simulink model "ADRCliju"  (R2024b)
settings: Solver=FixedStepAuto  StartTime=0.0  StopTime=20  RelTol=1e-3
undefined symbols (not defined in the file or in its folder): sigbuilder_block
libraries: spsPermanentMagnetSynchronousMachineLib x2, slpidlib x2, simulink x2, powerlib_extras x2, Solver_SF x1, spsDCVoltageSourceLib x1, spsUniversalBridgeLib x1, spspowerguiLib x1
settings Model: Creator=Dell  LastModifiedBy=L大锤
settings SolverCC: AlgebraicLoopSolver=TrustRegion
settings DataIOCC: ReturnWorkspaceOutputs=off
settings DebuggingCC: UnconnectedInputMsg=warning  UnconnectedOutputMsg=warning  UnconnectedLineMsg=warning  ArithmeticOperatorsInVariantConditions=warning
settings ModelReferenceCC: EnableRefExpFcnMdlSchedulingChecks=on
settings SFSimCC: CustomCodeUndefinedFunction=UseInterfaceOnly
settings RTWCC: GPUComputeCapability=3.5

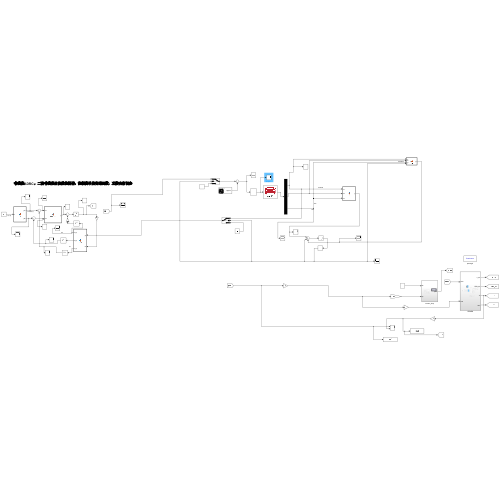
[thumbnail: Simulink's stored preview of the top-level diagram]
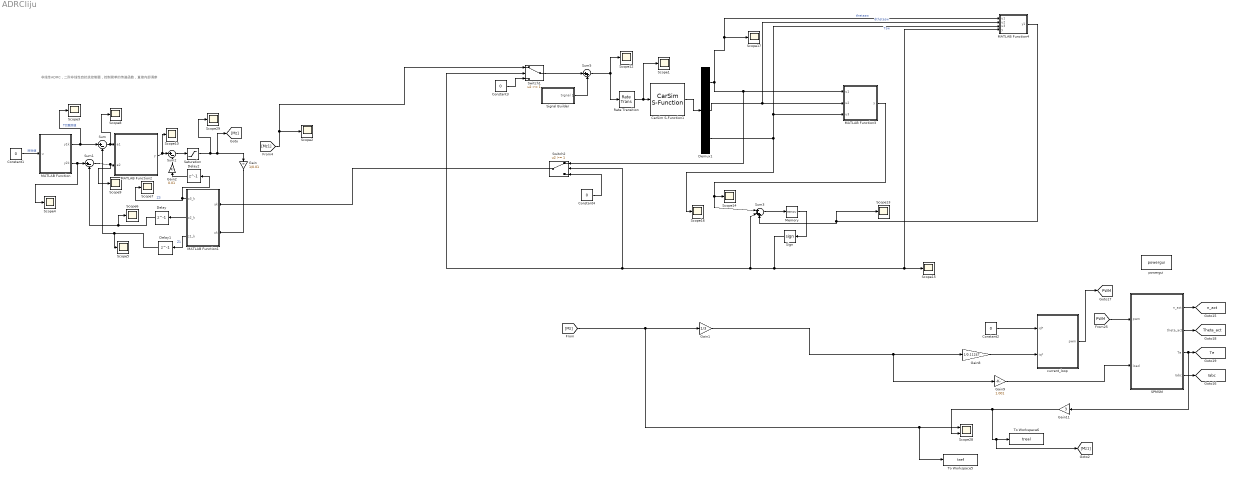
== system ADRCliju ==
  note: 非线性ADRC，二阶非线性自抗扰控制器，控制简单的传递函数，直接内部调参
  CarSim S-Function1 : Solver_SF/CarSim S-Function  Priority=1  SIMFILE=simfile.sim  Run_RTs=off  vs_state_ind=Run  StopMode_ind=Vehicle Model
  Constant{1..4} (4 alike) : Constant  Value=0
  Delay : Delay  DelayLength=1
  Delay1 : Delay  DelayLength=1
  Delay2 : Delay  DelayLength=1
  Demux1 : Demux  Outputs=3
  Gain : Gain  Gain=1/0.01
  Gain1 : Gain  Gain=1/3
  Gain11 : Gain  Gain=3
  Gain2 : Gain  Gain=0.01
  Gain8 : Gain  Gain=1/0.11247
  Gain9 : Gain  Gain=1.001
  MATLAB Function : MATLAB Function  TreatAsAtomicUnit=on
  MATLAB Function1 : MATLAB Function  TreatAsAtomicUnit=on
  MATLAB Function2 : MATLAB Function  TreatAsAtomicUnit=on
  MATLAB Function3 : MATLAB Function  TreatAsAtomicUnit=on
  MATLAB Function4 : MATLAB Function  TreatAsAtomicUnit=on
  Memory : Memory
  Rate Transition : RateTransition  OutPortSampleTime=1e-5
  SPMSM : Subsystem
  Saturation : Saturate  UpperLimit=2.99  LowerLimit=-2.99
  Scope{1..10,12..17,29} (17 alike) : Scope
  Scope28 : Scope  NumInputPorts=2
  Sign : Signum
  Signal Builder : Subsystem  Tag=STV Subsys  LoadFcn=sigbuilder_block('load');  StartFcn=sigbuilder_block('start');  StopFcn=sigbuilder_block('stop');  ClipboardFcn=sigbuilder_block('clipboard');  mask(Sigbuilder block){tuvar=[0:10]}
      mask help: Simulink:masks:SigbuilderBlock_MD
      mask init:
      | if ~strcmp(get_param(bdroot(gcbh),'SimulationStatus'),'stopped') tuvar = sigbuilder_block('maskInit'); end
      settings: CopyFcn=sigbuilder_block('copy');  DeleteFcn=sigbuilder_block('delete');  ModelCloseFcn=sigbuilder_block('modelClose');  PreSaveFcn=sigbuilder_block('preSave');  PauseFcn=sigbuilder_block('pause');  ContinueFcn=sigbuilder_block('continue');  NameChangeFcn=sigbuilder_block('namechange');  OpenFcn=sigbuilder_block('open',[437.6 186.6 550.4 400.2 ]);  CloseFcn=sigbuilder_block('close');
      mask Display: plot(0, 0, 100, 100,[2, 2, 32, 32, 2], [68, 8, 8, 68, 68],[32, 2], [38, 38], [32, 19, 2],[53, 60, 44], [32, 17, 17, 2],[16, 16, 31, 31]);txt = getActiveGroup(gcbh);text(2, 100, txt,'verticalAlignment', 'top');
  Sum : Sum  Inputs=|+-
  Sum1 : Sum  Inputs=|+-
  Sum2 : Sum  Inputs=|+-
  Sum3 : Sum  Inputs=|+++
  Sum5 : Sum  Inputs=|++
  Switch1 : Switch  Threshold=1  SaturateOnIntegerOverflow=off  InputSameDT=off
  Switch2 : Switch  Threshold=1  SaturateOnIntegerOverflow=off  InputSameDT=off
  To Workspace5 : ToWorkspace  VariableName=tref  SampleTime=-1
  To Workspace6 : ToWorkspace  VariableName=treal  SampleTime=-1
  current_loop : Subsystem
  powergui : spspowerguiLib/powergui  Priority=1  SimulationMode=Continuous  SampleTime=1/2000/500  frequency=60  Iterations=50  frequencyindice=0  Pbase=100e6  ErrMax=1e-4  UnitsV=kV  UnitsW=MW  buscounter=0  FunctionMessages=off  echomessages=off  EnableUseOfTLC=off  CurrentSourceSwitches=off  DisableSnubberDevices=off  DisableRonSwitches=off  DisableVfSwitches=off  DisplayEquations=off  AutomaticDiscreteSolvers=off  SolverType=Tustin/Backward Euler (TBE)  Interpol=off  ExternalGateDelay=off  methode=off  Ts=100  x0status=blocks  SPID=on  SwTol=0  HookPort=off  NonlinearTolerance=1e-4  nMaxIteration=100  ContinueOnMaxIteration=off  RestoreLinks=warning  ResistiveCurrentMeasurement=off  Frange=[0:2:500]  Ylog=off  Xlog=on  ShowGrid=off  save=off  variable=ZData  structure=ia  ZoomFFT=off  StartTime=.775  cycles=1  DisplayStyle=1  fundamental=400  FreqAxis=off  MaxFrequency=40000  frequencyindicesteady=1  RmsSteady=1  display=off
  tag scope: Iabc=global, PWM=global, Te=global, Theta_act=global, n_act=global
  wires:
  Constant1/1 -> MATLAB Function/1(u)  "目标值"
  Sum/1 -> Scope8/1, MATLAB Function2/1(e1)
  MATLAB Function/2(y2k) -> Scope4/1, Sum1/1
  Sum1/1 -> Scope9/1, MATLAB Function2/2(e2)
  MATLAB Function/1(y1k) -> Scope3/1, Sum/1  "TD跟踪值"
  Gain2/1 -> Sum2/2
  MATLAB Function1/1(z3_k) -> Scope7/1, Delay2/1  "Z3"
  MATLAB Function2/1(y) -> Scope10/1, Sum2/1
  Gain/1 -> MATLAB Function1/2(uk)
  MATLAB Function1/2(z2_k) -> Delay/1
  Delay/1 -> Scope6/1, Sum1/2
  Delay2/1 -> Gain2/1
  MATLAB Function1/3(z1_k) -> Delay1/1  "Z1"
  Delay1/1 -> Scope5/1, Sum/2
  Sum2/1 -> Saturation/1
  Saturation/1 -> Scope29/1, Gain/1, [Mz]
  [Mz] -> To Workspace5/1, Scope28/1, Gain1/1
  SPMSM/3(Te) -> Gain11/1, [Te]
  SPMSM/1(n_act) -> [n_act]
  [PWM] -> SPMSM/1(pwm)
  Constant2/1 -> current_loop/1(id*)
  Gain9/1 -> SPMSM/2(load)
  Gain8/1 -> current_loop/2(iq*)
  Gain11/1 -> [Mz1], To Workspace6/1, Scope28/2
  current_loop/1(pwm) -> [PWM]
  SPMSM/2(theta_act) -> [Theta_act]
  SPMSM/4(Iabc) -> [Iabc]
  Gain1/1 -> Gain9/1, Gain8/1
  Signal Builder/1(Signal 1) -> Sum5/2
  Switch2/1 -> MATLAB Function1/1(yk)
  CarSim S-Function1/1 -> Demux1/1
  Constant4/1 -> Switch2/3
  Sum5/1 -> Rate Transition/1, Scope12/1
  MATLAB Function3/1(y) -> Sum3/1, Scope14/1
  Demux1/1 -> Scope17/1, MATLAB Function4/1(u1), Switch2/1, MATLAB Function3/1(u1)  "thetasw"
  [Mz1] -> Switch1/1, Scope2/1
  Sign/1 -> Switch1/2, Switch2/2, Sum3/2, MATLAB Function4/4(y), Scope15/1
  Sum3/1 -> Memory/1
  MATLAB Function4/1(y1) -> Scope13/1, Sum3/3
  Demux1/2 -> MATLAB Function4/2(u2), MATLAB Function3/2(u2)  "dthstasw"
  Constant3/1 -> Switch1/3
  Memory/1 -> Sign/1
  Switch1/1 -> Sum5/1
  Demux1/3 -> MATLAB Function3/3(u3), MATLAB Function4/3(u3), Scope16/1  "Tsw"
  Rate Transition/1 -> CarSim S-Function1/1, Scope1/1

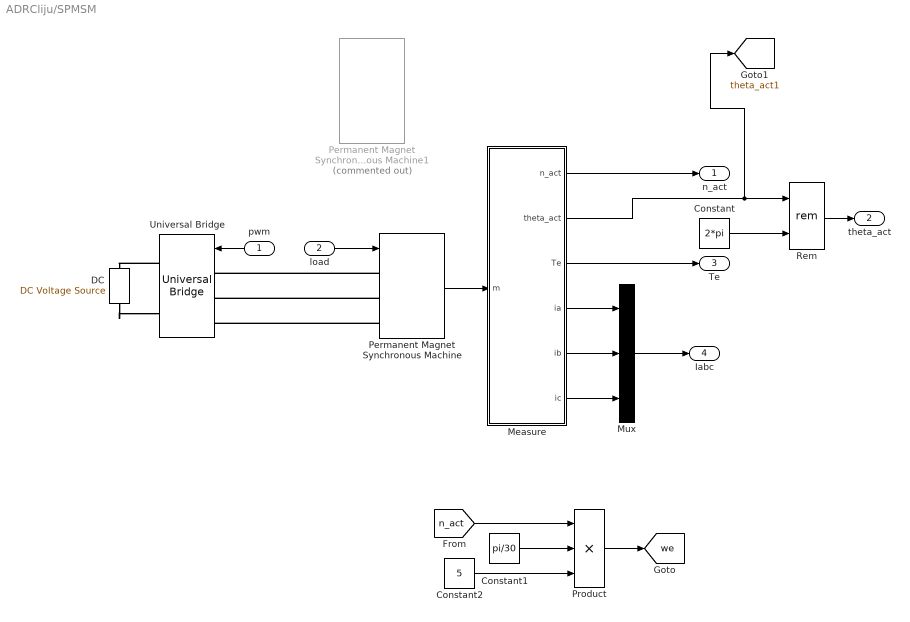
== system ADRCliju/SPMSM ==
  pwm : Inport
  load : Inport  Port=2
  Constant : Constant  Value=2*pi
  Constant1 : Constant  Value=pi/30
  Constant2 : Constant  Value=5
  "DC " : spsDCVoltageSourceLib/DC Voltage Source  Amplitude=200  Measurements=None
  Measure : Subsystem
  Mux : Mux  Inputs=3
  Permanent Magnet Synchronous Machine : spsPermanentMagnetSynchronousMachineLib/Permanent Magnet Synchronous Machine  NbPhases=3  FluxDistribution=Sinusoidal  RotorType=Round  MechanicalLoad=Torque Tm  PresetModel=No  ShowDetailedParameters=on  MeasurementBus=off  Resistance=0.12  Inductance=8.5e-3  dqInductances=[4e-3, 4e-3]  La=0.97e-3  MachineConstant=Voltage Constant (V_peak L-L / krpm)  Flux=0.014996  VoltageCst=13.6  TorqueCst=0.11247  Flat=120  Mechanical=[0.00107 0 5 0]  PolePairs=4  InitialConditions=[0,0, 0,0]  InitialConditions5ph=[0 0 0 0 0 0]  RefAngle=Aligned with phase A axis (original Park)  IterativeDiscreteModel=Trapezoidal non iterative  TsBlock=-1  TsPowergui=0
  Permanent Magnet Synchronous Machine1 : spsPermanentMagnetSynchronousMachineLib/Permanent Magnet Synchronous Machine  Commented=on  NbPhases=3  FluxDistribution=Sinusoidal  RotorType=Salient-pole  MechanicalLoad=Torque Tm  PresetModel=No  ShowDetailedParameters=on  MeasurementBus=off  Resistance=2.875  Inductance=8.5e-3  dqInductances=[4e-3, 4e-3]  La=0.000835  MachineConstant=Flux linkage established by magnets (V.s)  Flux=0.175  VoltageCst=126.966  TorqueCst=1.05  Flat=120  Mechanical=[0.003 0 4 0]  PolePairs=4  InitialConditions=[0,0, 0,0]  InitialConditions5ph=[0 0 0 0 0 0]  RefAngle=Aligned with phase A axis (original Park)  IterativeDiscreteModel=Trapezoidal non iterative  TsBlock=-1  TsPowergui=0
  Product : Product  Inputs=3
  Rem : Math  Operator=rem
  Universal Bridge : spsUniversalBridgeLib/Universal Bridge  Arms=3  SnubberResistance=1e5  SnubberCapacitance=inf  Device=IGBT / Diodes  Ron=1e-3  Lon=0  ForwardVoltages="[  0  0  ]"  ForwardVoltage=0  GTOparameters=[ 10e-6 , 20e-6 ]  IGBTparameters=[ 1e-6 , 2e-6 ]  Measurements=None  Measurements_2=None  converterType=Rectifier
  n_act : Outport
  theta_act : Outport  Port=2
  Te : Outport  Port=3
  Iabc : Outport  Port=4
  tag scope: theta_act1=global, we=global
  wires:
  pwm/1 -> Universal Bridge/1
  load/1 -> Permanent Magnet Synchronous Machine/1
  Permanent Magnet Synchronous Machine/1 -> Measure/1(m)
  Measure/1(n_act) -> n_act/1
  Measure/3(Te) -> Te/1
  Measure/4(ia) -> Mux/1
  Measure/5(ib) -> Mux/2
  Measure/6(ic) -> Mux/3
  Mux/1 -> Iabc/1
  Rem/1 -> theta_act/1
  Constant/1 -> Rem/2
  Measure/2(theta_act) -> [theta_act1], Rem/1
  [n_act] -> Product/1
  Constant1/1 -> Product/2
  Constant2/1 -> Product/3
  Product/1 -> [we]
  connections:
  "DC "/LConn1 -- Universal Bridge/RConn2
  Universal Bridge/RConn1 -- "DC "/RConn1
  Permanent Magnet Synchronous Machine/LConn3 -- Universal Bridge/LConn3
  Permanent Magnet Synchronous Machine/LConn1 -- Universal Bridge/LConn1
  Permanent Magnet Synchronous Machine/LConn2 -- Universal Bridge/LConn2

== system ADRCliju/Signal Builder ==
  Demux : Demux  Tag=STV Demux  Outputs=1
      settings: DisplayOption=none
  FromWs : FromWorkspace  Tag=STV FromWs  VariableName=tuvar
      SigBuilderData=|
      | common.afterFinalStr = 'Extrapolate'
      | common.sampleTime = 0
      | dataSet.timeRange = [0 10]
      | dataSet.name = 'Group 1'
      | sbobj.Groups.Name = 'Group 1'
      | sbobj.Groups.Signals.Name = 'Signal 1'
      | sbobj.Groups.Signals.XData = [0 1 1 5 5 10]
      | sbobj.Groups.Signals.YData = [0 0 4 4 0 0]
  Signal 1 : Outport  Tag=STV Outport
  wires:
  Demux/1 -> Signal 1/1
  FromWs/1 -> Demux/1

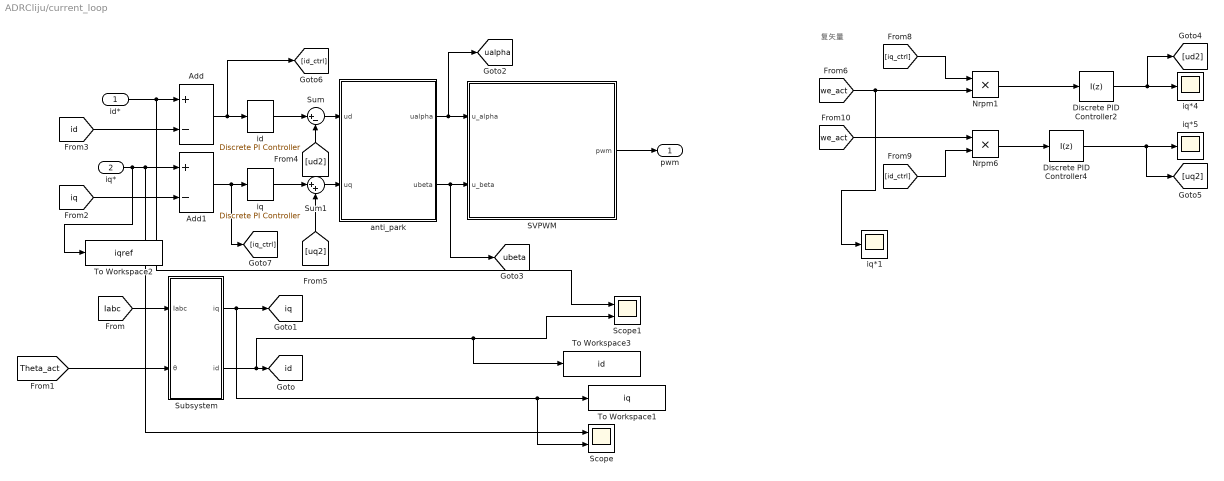
== system ADRCliju/current_loop ==
  note: 复矢量
  id* : Inport
  iq* : Inport  Port=2
  Add : Sum  Inputs=+-
  Add1 : Sum  Inputs=+-
  Discrete PID Controller2 : slpidlib/PID Controller  Controller=I  Form=Parallel  TimeDomain=Discrete-time  UseExternalTs=off  SampleTime=1e-4  IntegratorMethod=Forward Euler  FilterMethod=Forward Euler  ControllerParametersSource=internal  P=0  I=0.32/10000  UseKiTs=off  D=0  UseExternalDerivativeSource=off  N=100  UseFilter=on  TunerSelectOption=Transfer Function Based (PID Tuner App)  InitialConditionSource=internal  InitialConditionForIntegrator=0  InitialConditionForFilter=0  DifferentiatorICPrevScaledInput=0  ExternalReset=none  TrackingMode=off  Kt=1  LimitOutput=on  SatLimitsSource=internal  UpperSaturationLimit=600  LowerSaturationLimit=-600  LinearizeAsGain=off  AntiWindupMode=none  Kb=1  LimitIntegrator=off  UpperIntegratorSaturationLimit=inf  LowerIntegratorSaturationLimit=-inf  POutMin=[]  POutMax=[]  IOutMin=[]  IOutMax=[]  DOutMin=[]  DOutMax=[]  NOutMin=[]  NOutMax=[]  SumOutMin=[]  SumOutMax=[]  SaturationOutMin=[]  SaturationOutMax=[]  PParamMin=[]  PParamMax=[]  IParamMin=[]  IParamMax=[]  DParamMin=[]  DParamMax=[]  NParamMin=[]  NParamMax=[]  KbParamMin=[]  KbParamMax=[]  KtParamMin=[]  KtParamMax=[]  KbOutMin=[]  KbOutMax=[]  KtOutMin=[]  KtOutMax=[]  IntegratorOutMin=[]  IntegratorOutMax=[]  FilterOutMin=[]  FilterOutMax=[]  SumI1OutMin=[]  SumI1OutMax=[]  SumI2OutMin=[]  SumI2OutMax=[]  SumI3OutMin=[]  SumI3OutMax=[]  SumI4OutMin=[]  SumI4OutMax=[]  SumDOutMin=[]  SumDOutMax=[]  DifferentiatorOutMin=[]  DifferentiatorOutMax=[]  FilterDiffOutCoefMin=[]  FilterDiffOutCoefMax=[]  ReciprocalOutMin=[]  ReciprocalOutMax=[]  SumDenOutMin=[]  SumDenOutMax=[]  SumNumOutMin=[]  SumNumOutMax=[]  DivideOutMin=[]  DivideOutMax=[]  UdiffTsProdOutMin=[]  UdiffTsProdOutMax=[]  NTsProdOutMin=[]  NTsProdOutMax=[]  UintegralTsProdOutMin=[]  UintegralTsProdOutMax=[]  UngainTsProdOutMin=[]  UngainTsProdOutMax=[]  ClampingZeroOutDataTypeStr=Inherit: Inherit via back propagation  ClampingZeroOutMin=[]  ClampingZeroOutMax=[]  FilterDenConstantOutDataTypeStr=Inherit: Inherit via back propagation  FilterDenConstantOutMin=[]  FilterDenConstantOutMax=[]  PCopyOutDataTypeStr=Inherit: Inherit via back propagation  PCopyOutMin=[]  PCopyOutMax=[]  NCopyOutDataTypeStr=Inherit: Inherit via back propagation  NCopyOutMin=[]  NCopyOutMax=[]  IntegratorContinuousStateAttributes=''  IntegratorStateMustResolveToSignalObject=off  IntegratorRTWStateStorageClass=Auto  FilterContinuousStateAttributes=''  FilterStateMustResolveToSignalObject=off  FilterRTWStateStorageClass=Auto  ParallelPVariant=Disabled  IdealPVariant=Disabled  IVariant=InternalParameters  DVariant=Disabled  IntegratorVariant=Discrete  SatVariant=Enabled  AWVariant=Passthrough  PCopyVariant=Disabled  TRVariant=Disabled  FdbkBlocksVariant=Forward  IdealPFdbkVariant=Disabled  SatFdbkVariant=Disabled  DerivativeFilterVariant=Disabled  NVariant=Disabled  NCopyVariant=Disabled_SignalSpec  FilterICVariant=Disabled  IntegratorICVariant=InternalICs  ExternalResetVariant=Disabled  TRSumVariant=Passthrough  SumFdbkVariant=Disabled  SumVariant=Passthrough_I  TsampFilterVariant=InternalTs  TsampNgainVariant=Passthrough  TsampIntegralVariant=Disabled_SignalSpec  ExternalSaturationOutDataTypeStr=Inherit: Same as second input  DerivativeSourceVariant=Disabled  PreIntVariant=InternalPreInt
  Discrete PID Controller4 : slpidlib/PID Controller  Controller=I  Form=Parallel  TimeDomain=Discrete-time  UseExternalTs=off  SampleTime=1e-4  IntegratorMethod=Forward Euler  FilterMethod=Forward Euler  ControllerParametersSource=internal  P=0  I=0.32/10000  UseKiTs=off  D=0  UseExternalDerivativeSource=off  N=100  UseFilter=on  TunerSelectOption=Transfer Function Based (PID Tuner App)  InitialConditionSource=internal  InitialConditionForIntegrator=0  InitialConditionForFilter=0  DifferentiatorICPrevScaledInput=0  ExternalReset=none  TrackingMode=off  Kt=1  LimitOutput=on  SatLimitsSource=internal  UpperSaturationLimit=600  LowerSaturationLimit=-600  LinearizeAsGain=off  AntiWindupMode=none  Kb=1  LimitIntegrator=off  UpperIntegratorSaturationLimit=inf  LowerIntegratorSaturationLimit=-inf  POutMin=[]  POutMax=[]  IOutMin=[]  IOutMax=[]  DOutMin=[]  DOutMax=[]  NOutMin=[]  NOutMax=[]  SumOutMin=[]  SumOutMax=[]  SaturationOutMin=[]  SaturationOutMax=[]  PParamMin=[]  PParamMax=[]  IParamMin=[]  IParamMax=[]  DParamMin=[]  DParamMax=[]  NParamMin=[]  NParamMax=[]  KbParamMin=[]  KbParamMax=[]  KtParamMin=[]  KtParamMax=[]  KbOutMin=[]  KbOutMax=[]  KtOutMin=[]  KtOutMax=[]  IntegratorOutMin=[]  IntegratorOutMax=[]  FilterOutMin=[]  FilterOutMax=[]  SumI1OutMin=[]  SumI1OutMax=[]  SumI2OutMin=[]  SumI2OutMax=[]  SumI3OutMin=[]  SumI3OutMax=[]  SumI4OutMin=[]  SumI4OutMax=[]  SumDOutMin=[]  SumDOutMax=[]  DifferentiatorOutMin=[]  DifferentiatorOutMax=[]  FilterDiffOutCoefMin=[]  FilterDiffOutCoefMax=[]  ReciprocalOutMin=[]  ReciprocalOutMax=[]  SumDenOutMin=[]  SumDenOutMax=[]  SumNumOutMin=[]  SumNumOutMax=[]  DivideOutMin=[]  DivideOutMax=[]  UdiffTsProdOutMin=[]  UdiffTsProdOutMax=[]  NTsProdOutMin=[]  NTsProdOutMax=[]  UintegralTsProdOutMin=[]  UintegralTsProdOutMax=[]  UngainTsProdOutMin=[]  UngainTsProdOutMax=[]  ClampingZeroOutDataTypeStr=Inherit: Inherit via back propagation  ClampingZeroOutMin=[]  ClampingZeroOutMax=[]  FilterDenConstantOutDataTypeStr=Inherit: Inherit via back propagation  FilterDenConstantOutMin=[]  FilterDenConstantOutMax=[]  PCopyOutDataTypeStr=Inherit: Inherit via back propagation  PCopyOutMin=[]  PCopyOutMax=[]  NCopyOutDataTypeStr=Inherit: Inherit via back propagation  NCopyOutMin=[]  NCopyOutMax=[]  IntegratorContinuousStateAttributes=''  IntegratorStateMustResolveToSignalObject=off  IntegratorRTWStateStorageClass=Auto  FilterContinuousStateAttributes=''  FilterStateMustResolveToSignalObject=off  FilterRTWStateStorageClass=Auto  ParallelPVariant=Disabled  IdealPVariant=Disabled  IVariant=InternalParameters  DVariant=Disabled  IntegratorVariant=Discrete  SatVariant=Enabled  AWVariant=Passthrough  PCopyVariant=Disabled  TRVariant=Disabled  FdbkBlocksVariant=Forward  IdealPFdbkVariant=Disabled  SatFdbkVariant=Disabled  DerivativeFilterVariant=Disabled  NVariant=Disabled  NCopyVariant=Disabled_SignalSpec  FilterICVariant=Disabled  IntegratorICVariant=InternalICs  ExternalResetVariant=Disabled  TRSumVariant=Passthrough  SumFdbkVariant=Disabled  SumVariant=Passthrough_I  TsampFilterVariant=InternalTs  TsampNgainVariant=Passthrough  TsampIntegralVariant=Disabled_SignalSpec  ExternalSaturationOutDataTypeStr=Inherit: Same as second input  DerivativeSourceVariant=Disabled  PreIntVariant=InternalPreInt
  Nrpm1 : Product
  Nrpm6 : Product
  SVPWM : Subsystem
  Scope : Scope  NumInputPorts=2
  Scope1 : Scope  NumInputPorts=2
  Subsystem : Subsystem
  Sum : Sum  Inputs=|+-
  Sum1 : Sum  Inputs=|++
  To Workspace1 : ToWorkspace  VariableName=iq  SampleTime=-1
  To Workspace2 : ToWorkspace  VariableName=iqref  SampleTime=-1
  To Workspace3 : ToWorkspace  VariableName=id  SampleTime=-1
  anti_park : Subsystem
  id : powerlib_extras/Discrete  Control Blocks/Discrete PI Controller  Kp=0.32*2  Ki=0.004*2  Par_Limits=[200/1.732 -200/1.732]  Init=0  Ts=1e-4
  iq : powerlib_extras/Discrete  Control Blocks/Discrete PI Controller  Kp=0.32*2  Ki=0.004*2  Par_Limits=[200/1.732 -200/1.732]  Init=0  Ts=1e-4
  iq*1 : Scope
  iq*4 : Scope
  iq*5 : Scope
  pwm : Outport
  tag scope: id=global, iq=global, ualpha=global, ubeta=global
  wires:
  id*/1 -> Scope1/1, Add/1
  Add/1 -> [id_ctrl], id/1
  iq*/1 -> To Workspace2/1, Scope/1, Add1/1
  Add1/1 -> [iq_ctrl], iq/1
  anti_park/1(ualpha) -> [ualpha], SVPWM/1(u_alpha)
  anti_park/2(ubeta) -> [ubeta], SVPWM/2(u_beta)
  SVPWM/1(pwm) -> pwm/1
  [Iabc] -> Subsystem/1(Iabc)
  [iq] -> Add1/2
  [id] -> Add/2
  [Theta_act] -> Subsystem/2(θ)
  [ud2] -> Sum/2
  [uq2] -> Sum1/2
  id/1 -> Sum/1
  Sum/1 -> anti_park/1(ud)
  iq/1 -> Sum1/1
  Sum1/1 -> anti_park/2(uq)
  [id_ctrl] -> Nrpm6/2
  Nrpm1/1 -> Discrete PID Controller2/1
  Nrpm6/1 -> Discrete PID Controller4/1
  Discrete PID Controller2/1 -> [ud2], iq*4/1
  [we_act] -> iq*1/1, Nrpm1/2
  [we_act] -> Nrpm6/1
  Discrete PID Controller4/1 -> iq*5/1, [uq2]
  [iq_ctrl] -> Nrpm1/1
  Subsystem/2(id) -> To Workspace3/1, Scope1/2, [id]
  Subsystem/1(iq) -> To Workspace1/1, Scope/2, [iq]

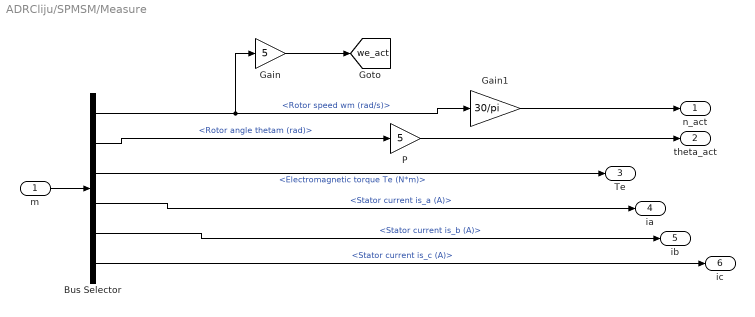
== system ADRCliju/SPMSM/Measure ==
  m : Inport
  Bus Selector : BusSelector  OutputSignals=Rotor speed wm (rad/s),Rotor angle thetam (rad),Electromagnetic torque Te (N*m),Stator current is_a (A),Stator current is_b (A),Stator current is_c (A)
  Gain : Gain  Gain=5
  Gain1 : Gain  Gain=30/pi
  P : Gain  Gain=5
  n_act : Outport  VectorParamsAs1DForOutWhenUnconnected=off
  theta_act : Outport  Port=2  VectorParamsAs1DForOutWhenUnconnected=off
  Te : Outport  Port=3  VectorParamsAs1DForOutWhenUnconnected=off
  ia : Outport  Port=4  VectorParamsAs1DForOutWhenUnconnected=off
  ib : Outport  Port=5  VectorParamsAs1DForOutWhenUnconnected=off
  ic : Outport  Port=6  VectorParamsAs1DForOutWhenUnconnected=off
  tag scope: we_act=global
  wires:
  m/1 -> Bus Selector/1
  Bus Selector/3 -> Te/1  "<Electromagnetic torque Te (N*m)>"
  Bus Selector/1 -> Gain/1, Gain1/1  "<Rotor speed wm (rad/s)>"
  Bus Selector/2 -> P/1  "<Rotor angle thetam (rad)>"
  Bus Selector/5 -> ib/1  "<Stator current is_b (A)>"
  Bus Selector/6 -> ic/1  "<Stator current is_c (A)>"
  P/1 -> theta_act/1
  Gain1/1 -> n_act/1
  Bus Selector/4 -> ia/1  "<Stator current is_a (A)>"
  Gain/1 -> [we_act]

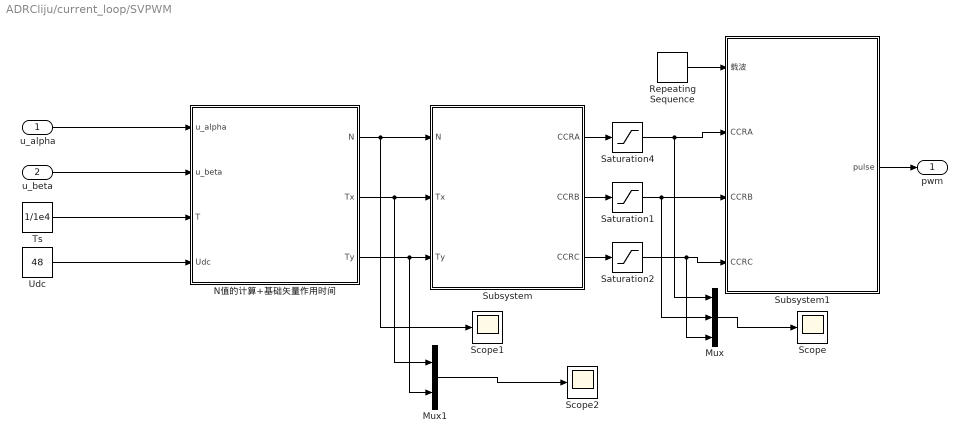
== system ADRCliju/current_loop/SVPWM ==
  u_alpha : Inport
  u_beta : Inport  Port=2
  Mux : Mux  Inputs=3
  Mux1 : Mux  Inputs=2
  N值的计算+基础矢量作用时间 : Subsystem
  Repeating Sequence : simulink/Sources/Repeating Sequence  rep_seq_t=[0 1/1e4/2 1/1e4]  rep_seq_y=[0 1/1e4/2 0]
  Saturation1 : Saturate  UpperLimit=1/1e4/2  LowerLimit=0
  Saturation2 : Saturate  UpperLimit=1/1e4/2  LowerLimit=0
  Saturation4 : Saturate  UpperLimit=1/1e4/2  LowerLimit=0
  Scope : Scope
  Scope1 : Scope
  Scope2 : Scope
  Subsystem : Subsystem
  Subsystem1 : Subsystem
  Ts : Constant  Value=1/1e4
  Udc : Constant  Value=48
  pwm : Outport
  wires:
  Repeating Sequence/1 -> Subsystem1/1(载波)
  Subsystem1/1(pulse) -> pwm/1
  N值的计算+基础矢量作用时间/3(Ty) -> Mux1/2, Subsystem/3(Ty)
  N值的计算+基础矢量作用时间/2(Tx) -> Mux1/1, Subsystem/2(Tx)
  N值的计算+基础矢量作用时间/1(N) -> Scope1/1, Subsystem/1(N)
  Udc/1 -> N值的计算+基础矢量作用时间/4(Udc)
  Ts/1 -> N值的计算+基础矢量作用时间/3(T)
  u_beta/1 -> N值的计算+基础矢量作用时间/2(u_beta)
  u_alpha/1 -> N值的计算+基础矢量作用时间/1(u_alpha)
  Subsystem/2(CCRB) -> Saturation1/1
  Subsystem/3(CCRC) -> Saturation2/1
  Subsystem/1(CCRA) -> Saturation4/1
  Mux/1 -> Scope/1
  Saturation4/1 -> Mux/1, Subsystem1/2(CCRA)
  Saturation1/1 -> Mux/2, Subsystem1/3(CCRB)
  Saturation2/1 -> Mux/3, Subsystem1/4(CCRC)
  Mux1/1 -> Scope2/1

== system ADRCliju/current_loop/Subsystem ==
  Iabc : Inport
  θ : Inport  Port=2
  Clark : Subsystem
  Demux : Demux  Outputs=3
  "Park " : Subsystem
  iq : Outport  VectorParamsAs1DForOutWhenUnconnected=off
  id : Outport  Port=2  VectorParamsAs1DForOutWhenUnconnected=off
  tag scope: ialpha=global, ibeta=global
  wires:
  Demux/1 -> Clark/1(ia)
  Demux/3 -> Clark/3(ic)
  Demux/2 -> Clark/2(ib)
  Iabc/1 -> Demux/1
  θ/1 -> "Park "/3(Theta)
  Clark/2(ibeta) -> [ibeta], "Park "/2(ibeta)
  Clark/1(ialfa) -> [ialpha], "Park "/1(ialfa)
  "Park "/1(iq) -> iq/1
  "Park "/2(id) -> id/1

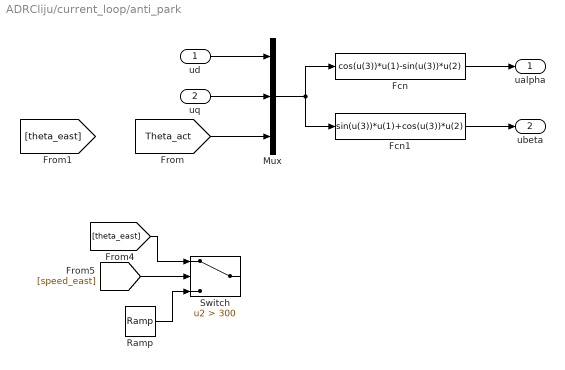
== system ADRCliju/current_loop/anti_park ==
  ud : Inport
  uq : Inport  Port=2
  Fcn : Fcn  Expr=cos(u(3))*u(1)-sin(u(3))*u(2)
  Fcn1 : Fcn  Expr=sin(u(3))*u(1)+cos(u(3))*u(2)
  Mux : Mux  Inputs=3
  Ramp : simulink/Sources/Ramp  slope=50  start=0  InitialOutput=0
  Switch : Switch  Criteria=u2 > Threshold  Threshold=300  SaturateOnIntegerOverflow=off  InputSameDT=off
  ualpha : Outport
  ubeta : Outport  Port=2
  wires:
  Fcn/1 -> ualpha/1
  ud/1 -> Mux/1
  uq/1 -> Mux/2
  Fcn1/1 -> ubeta/1
  Mux/1 -> Fcn/1, Fcn1/1
  [theta_east] -> Switch/1
  Ramp/1 -> Switch/3
  [speed_east] -> Switch/2
  [Theta_act] -> Mux/3

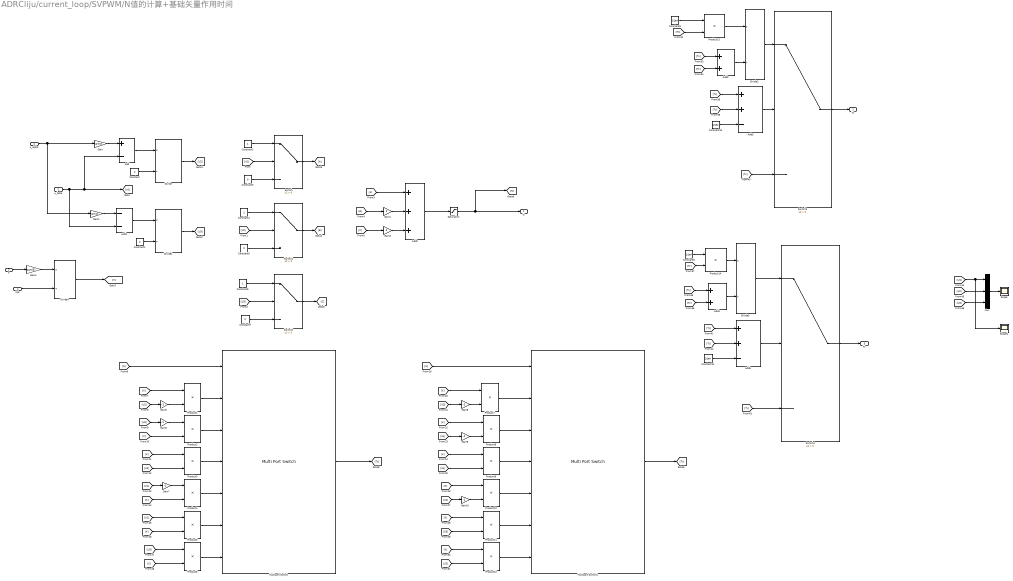
== system ADRCliju/current_loop/SVPWM/N值的计算+基础矢量作用时间 ==
  u_alpha : Inport
  u_beta : Inport  Port=2
  T : Inport  Port=3
  Udc : Inport  Port=4
  Add : Sum  Inputs=+-
  Add1 : Sum  Inputs=--
  Add2 : Sum  Inputs=+++
  Add3 : Sum
  Add4 : Sum
  Add5 : Sum  Inputs=++-
  Add6 : Sum  Inputs=++-
  Constant : Constant  Value=2
  Constant1 : Constant  Value=2
  Constant{8..11} (4 alike) : Constant  Value=1/1e4
  Constant2 : Constant
  Constant3 : Constant  Value=0
  Constant4 : Constant
  Constant5 : Constant  Value=0
  Constant6 : Constant
  Constant7 : Constant  Value=0
  Divide{,1..4} (5 alike) : Product  Inputs=*/
  From3 : From
  Gain : Gain  Gain=sqrt(3)
  Gain1 : Gain  Gain=2
  Gain{5..10} (6 alike) : Gain  Gain=-1
  Gain2 : Gain  Gain=sqrt(3)
  Gain3 : Gain  Gain=4
  Gain4 : Gain  Gain=sqrt(3)
  Goto3 : Goto
  Multiport Switch : MultiPortSwitch  Inputs=6  SaturateOnIntegerOverflow=off  InputSameDT=off
  Multiport Switch1 : MultiPortSwitch  Inputs=6  SaturateOnIntegerOverflow=off  InputSameDT=off
  Mux : Mux  Inputs=3
  Product{1..14} (14 alike) : Product
  Saturation : Saturate  UpperLimit=6  LowerLimit=1
  Scope : Scope
  Scope1 : Scope
  Switch{,1..4} (5 alike) : Switch  Criteria=u2 > Threshold  SaturateOnIntegerOverflow=off  InputSameDT=off
  N : Outport
  Tx : Outport  Port=2
  Ty : Outport  Port=3
  wires:
  Switch4/1 -> Ty/1
  [Ty] -> Switch4/3
  Constant11/1 -> Add6/3
  [Ty] -> Add6/2
  [Tx] -> Add6/1
  Add6/1 -> Switch4/2
  Divide3/1 -> Switch4/1
  Switch3/1 -> Tx/1
  [Tx] -> Switch3/3
  Constant10/1 -> Add5/3
  [Ty] -> Add5/2
  [Tx] -> Add5/1
  Add5/1 -> Switch3/2
  Divide2/1 -> Switch3/1
  [Ty] -> Product14/2
  Constant9/1 -> Product14/1
  Product14/1 -> Divide3/1
  [Tx] -> Add4/1
  [Ty] -> Add4/2
  Add4/1 -> Divide3/2
  [Ty] -> Add3/2
  [Tx] -> Add3/1
  Add3/1 -> Divide2/2
  [Tx] -> Product13/2
  Constant8/1 -> Product13/1
  Product13/1 -> Divide2/1
  [U2] -> Product12/2
  [K] -> Product12/1
  Product12/1 -> Multiport Switch1/7
  [U3] -> Product11/2
  [K] -> Product11/1
  Product11/1 -> Multiport Switch1/6
  Gain10/1 -> Product10/2
  [U2] -> Gain10/1
  [K] -> Product10/1
  Product10/1 -> Multiport Switch1/5
  [U1] -> Product9/2
  [K] -> Product9/1
  Product9/1 -> Multiport Switch1/4
  Gain9/1 -> Product8/2
  [U1] -> Gain9/1
  [K] -> Product8/1
  Product8/1 -> Multiport Switch1/3
  Multiport Switch1/1 -> [Ty]
  Gain8/1 -> Product7/2
  [U3] -> Gain8/1
  [K] -> Product7/1
  Product7/1 -> Multiport Switch1/2
  [N] -> Multiport Switch1/1
  [K] -> Product6/2
  [U3] -> Product6/1
  Product6/1 -> Multiport Switch/7
  [K] -> Product5/2
  [U1] -> Product5/1
  Product5/1 -> Multiport Switch/6
  [K] -> Product4/2
  [U1] -> Gain7/1
  Gain7/1 -> Product4/1
  Product4/1 -> Multiport Switch/5
  [U2] -> Product3/2
  [K] -> Product3/1
  Product3/1 -> Multiport Switch/4
  [K] -> Product2/2
  Gain6/1 -> Product2/1
  [U3] -> Gain6/1
  Gain5/1 -> Product1/2
  Product2/1 -> Multiport Switch/3
  Multiport Switch/1 -> [Tx]
  [U2] -> Gain5/1
  [K] -> Product1/1
  Product1/1 -> Multiport Switch/2
  Udc/1 -> Divide4/2
  T/1 -> Gain4/1
  Gain4/1 -> Divide4/1
  Divide4/1 -> [K]
  [N] -> Multiport Switch/1
  Saturation/1 -> N/1, [N]
  Add2/1 -> Saturation/1
  [C] -> Gain3/1
  Gain3/1 -> Add2/3
  [B] -> Gain1/1
  Gain1/1 -> Add2/2
  From3/1 -> Add2/1
  Switch2/1 -> [C]
  Constant7/1 -> Switch2/3
  Constant6/1 -> Switch2/1
  [U3] -> Switch2/2
  Switch1/1 -> [B]
  Constant5/1 -> Switch1/3
  Constant4/1 -> Switch1/1
  [U2] -> Switch1/2
  Constant3/1 -> Switch/3
  Constant2/1 -> Switch/1
  Switch/1 -> Goto3/1
  [U1] -> Switch/2
  u_beta/1 -> [U1], Add/2, Add1/2
  Gain2/1 -> Add1/1
  Divide1/1 -> [U3]
  Constant1/1 -> Divide1/2
  Add1/1 -> Divide1/1
  Divide/1 -> [U2]
  Constant/1 -> Divide/2
  Add/1 -> Divide/1
  u_alpha/1 -> Gain/1, Gain2/1
  Gain/1 -> Add/1
  [U1] -> Scope1/1, Mux/1
  [U2] -> Mux/2
  [U3] -> Mux/3
  Mux/1 -> Scope/1

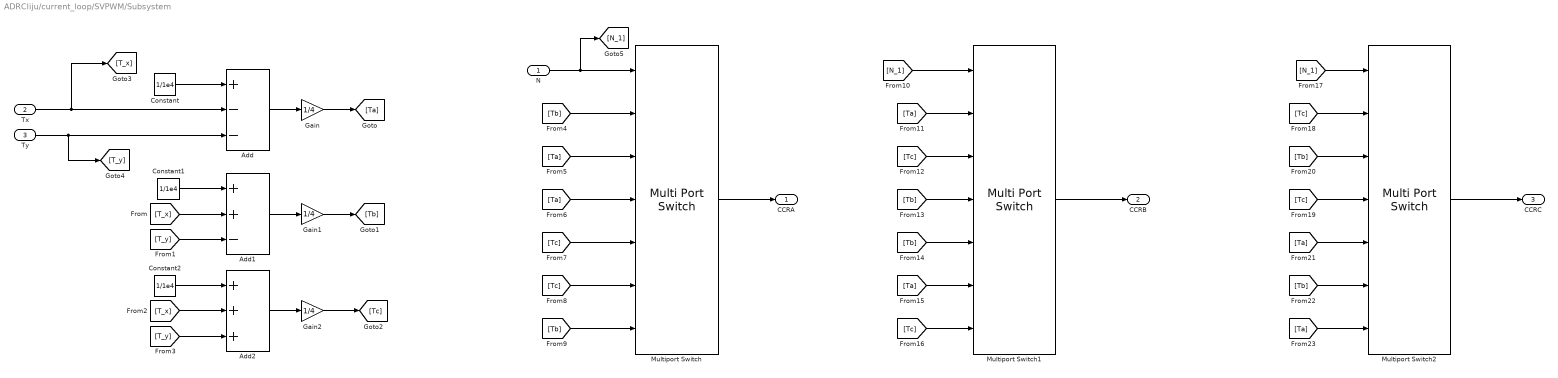
== system ADRCliju/current_loop/SVPWM/Subsystem ==
  N : Inport
  Tx : Inport  Port=2
  Ty : Inport  Port=3
  Add : Sum  Inputs=+--
  Add1 : Sum  Inputs=++-
  Add2 : Sum  Inputs=+++
  Constant : Constant  Value=1/1e4
  Constant1 : Constant  Value=1/1e4
  Constant2 : Constant  Value=1/1e4
  Gain : Gain  Gain=1/4
  Gain1 : Gain  Gain=1/4
  Gain2 : Gain  Gain=1/4
  Multiport Switch : MultiPortSwitch  Inputs=6  SaturateOnIntegerOverflow=off  InputSameDT=off
  Multiport Switch1 : MultiPortSwitch  Inputs=6  SaturateOnIntegerOverflow=off  InputSameDT=off
  Multiport Switch2 : MultiPortSwitch  Inputs=6  SaturateOnIntegerOverflow=off  InputSameDT=off
  CCRA : Outport
  CCRB : Outport  Port=2
  CCRC : Outport  Port=3
  wires:
  [Ta] -> Multiport Switch2/7
  [Tb] -> Multiport Switch2/6
  [Ta] -> Multiport Switch2/5
  [Tc] -> Multiport Switch2/4
  [Tb] -> Multiport Switch2/3
  [Tc] -> Multiport Switch2/2
  Multiport Switch2/1 -> CCRC/1
  [N_1] -> Multiport Switch2/1
  [Tc] -> Multiport Switch1/7
  [Ta] -> Multiport Switch1/6
  [Tb] -> Multiport Switch1/5
  [Tb] -> Multiport Switch1/4
  [Tc] -> Multiport Switch1/3
  [Ta] -> Multiport Switch1/2
  Multiport Switch1/1 -> CCRB/1
  [N_1] -> Multiport Switch1/1
  [Tb] -> Multiport Switch/7
  [Tc] -> Multiport Switch/6
  [Tc] -> Multiport Switch/5
  [Ta] -> Multiport Switch/4
  [Ta] -> Multiport Switch/3
  [Tb] -> Multiport Switch/2
  Multiport Switch/1 -> CCRA/1
  N/1 -> Multiport Switch/1, [N_1]
  [T_y] -> Add2/3
  [T_x] -> Add2/2
  Constant2/1 -> Add2/1
  Gain2/1 -> [Tc]
  Add2/1 -> Gain2/1
  Gain1/1 -> [Tb]
  Add1/1 -> Gain1/1
  [T_y] -> Add1/3
  [T_x] -> Add1/2
  Constant1/1 -> Add1/1
  Gain/1 -> [Ta]
  Add/1 -> Gain/1
  Ty/1 -> Add/3, [T_y]
  Tx/1 -> Add/2, [T_x]
  Constant/1 -> Add/1

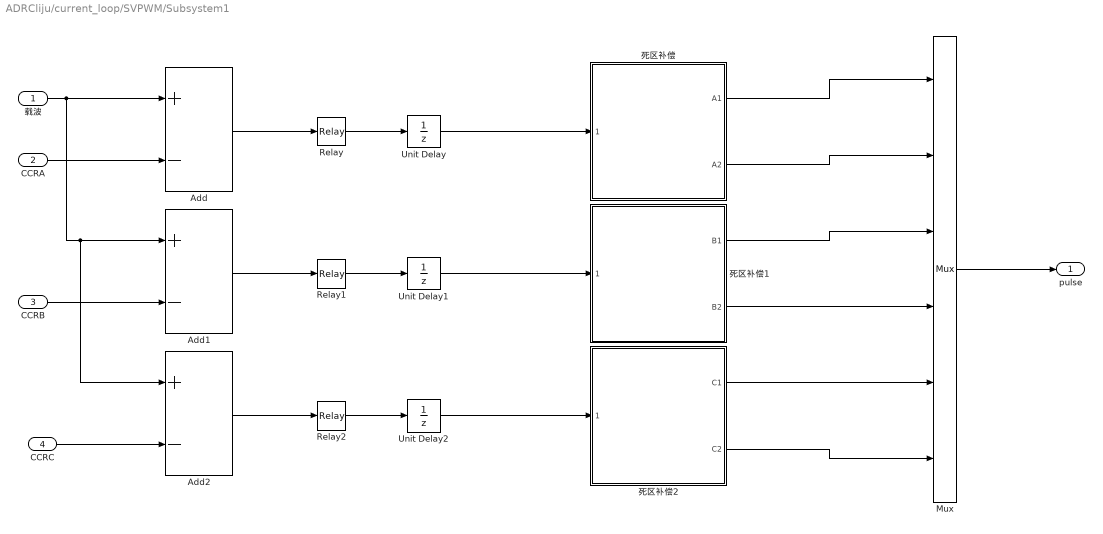
== system ADRCliju/current_loop/SVPWM/Subsystem1 ==
  载波 : Inport
  CCRA : Inport  Port=2
  CCRB : Inport  Port=3
  CCRC : Inport  Port=4
  Add : Sum  Inputs=+-
  Add1 : Sum  Inputs=+-
  Add2 : Sum  Inputs=+-
  Mux : Mux  Inputs=6
  Relay : Relay
  Relay1 : Relay
  Relay2 : Relay
  Unit Delay : UnitDelay  SampleTime=-1  HasFrameUpgradeWarning=on
  Unit Delay1 : UnitDelay  SampleTime=-1  HasFrameUpgradeWarning=on
  Unit Delay2 : UnitDelay  SampleTime=-1  HasFrameUpgradeWarning=on
  死区补偿 : Subsystem
  死区补偿1 : Subsystem
  死区补偿2 : Subsystem
  pulse : Outport
  wires:
  Mux/1 -> pulse/1
  死区补偿2/2(C2) -> Mux/6
  死区补偿2/1(C1) -> Mux/5
  死区补偿1/2(B2) -> Mux/4
  死区补偿1/1(B1) -> Mux/3
  死区补偿/2(A2) -> Mux/2
  死区补偿/1(A1) -> Mux/1
  Unit Delay2/1 -> 死区补偿2/1(1)
  Unit Delay1/1 -> 死区补偿1/1(1)
  Unit Delay/1 -> 死区补偿/1(1)
  Relay2/1 -> Unit Delay2/1
  Relay1/1 -> Unit Delay1/1
  Relay/1 -> Unit Delay/1
  Add2/1 -> Relay2/1
  Add1/1 -> Relay1/1
  Add/1 -> Relay/1
  CCRC/1 -> Add2/2
  CCRB/1 -> Add1/2
  CCRA/1 -> Add/2
  载波/1 -> Add/1, Add1/1, Add2/1

== system ADRCliju/current_loop/Subsystem/Clark ==
  ia : Inport
  ib : Inport  Port=2
  ic : Inport  Port=3
  Fcn : Fcn  Expr=2/3*(u[1]-0.5*u[2]-0.5*u[3])
  Fcn1 : Fcn  Expr=2/3*(sqrt(3/4)*u(2)-sqrt(3/4)*u(3))
  Mux : Mux  Inputs=3
  ialfa : Outport  VectorParamsAs1DForOutWhenUnconnected=off
  ibeta : Outport  Port=2  VectorParamsAs1DForOutWhenUnconnected=off
  wires:
  ic/1 -> Mux/3
  Fcn1/1 -> ibeta/1
  Fcn/1 -> ialfa/1
  Mux/1 -> Fcn1/1, Fcn/1
  ib/1 -> Mux/2
  ia/1 -> Mux/1

== system ADRCliju/current_loop/Subsystem/Park  ==
  ialfa : Inport
  ibeta : Inport  Port=2
  Theta : Inport  Port=3
  Fcn : Fcn  Expr=u(2)*cos(u(3))-u(1)*sin(u(3))
  Fcn1 : Fcn  Expr=u(2)*sin(u(3))+u(1)*cos(u(3))
  Mux : Mux  Inputs=3
  iq : Outport  VectorParamsAs1DForOutWhenUnconnected=off
  id : Outport  Port=2  VectorParamsAs1DForOutWhenUnconnected=off
  wires:
  Theta/1 -> Mux/3
  Fcn1/1 -> id/1
  Fcn/1 -> iq/1
  Mux/1 -> Fcn/1, Fcn1/1
  ibeta/1 -> Mux/2
  ialfa/1 -> Mux/1

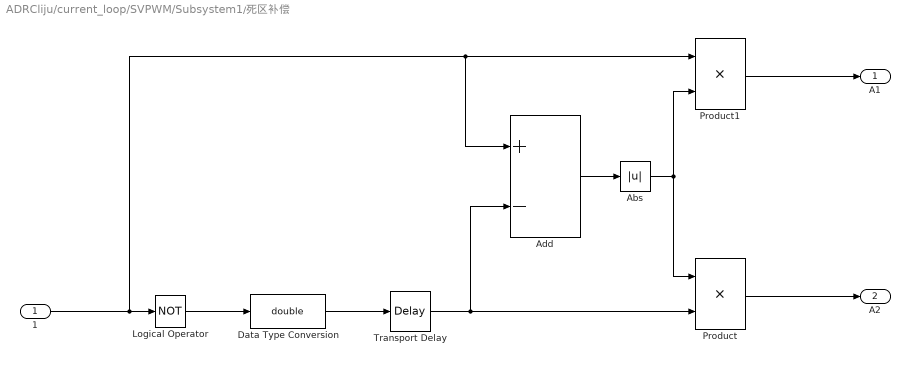
== system ADRCliju/current_loop/SVPWM/Subsystem1/死区补偿 ==
  1 : Inport
  Abs : Abs  SaturateOnIntegerOverflow=off
  Add : Sum  Inputs=+-
  Data Type Conversion : DataTypeConversion  OutDataTypeStr=double  SaturateOnIntegerOverflow=off  RndMeth=Floor
  Logical Operator : Logic  Operator=NOT  AllPortsSameDT=off  OutDataTypeStr=boolean
  Product : Product
  Product1 : Product
  Transport Delay : TransportDelay  DelayTime=0
  A1 : Outport
  A2 : Outport  Port=2
  wires:
  Abs/1 -> Product1/2, Product/1
  Product1/1 -> A1/1
  Add/1 -> Abs/1
  Product/1 -> A2/1
  Transport Delay/1 -> Product/2, Add/2
  Data Type Conversion/1 -> Transport Delay/1
  Logical Operator/1 -> Data Type Conversion/1
  1/1 -> Logical Operator/1, Add/1, Product1/1

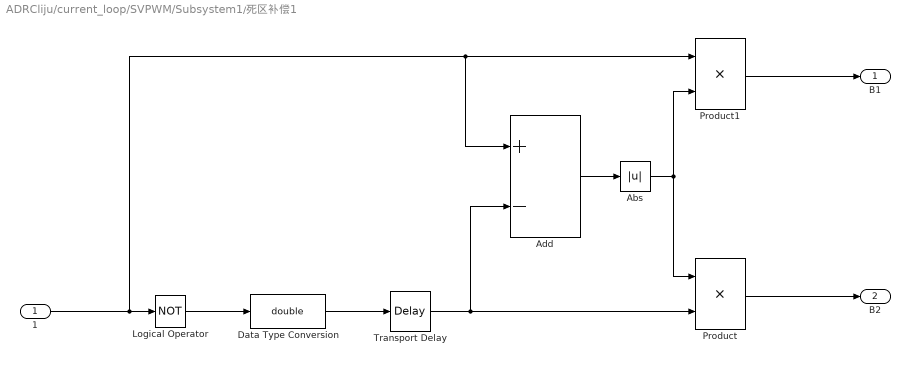
== system ADRCliju/current_loop/SVPWM/Subsystem1/死区补偿1 ==
  1 : Inport
  Abs : Abs  SaturateOnIntegerOverflow=off
  Add : Sum  Inputs=+-
  Data Type Conversion : DataTypeConversion  OutDataTypeStr=double  SaturateOnIntegerOverflow=off  RndMeth=Floor
  Logical Operator : Logic  Operator=NOT  AllPortsSameDT=off  OutDataTypeStr=boolean
  Product : Product
  Product1 : Product
  Transport Delay : TransportDelay  DelayTime=0
  B1 : Outport
  B2 : Outport  Port=2
  wires:
  1/1 -> Product1/1, Add/1, Logical Operator/1
  Logical Operator/1 -> Data Type Conversion/1
  Data Type Conversion/1 -> Transport Delay/1
  Transport Delay/1 -> Add/2, Product/2
  Product/1 -> B2/1
  Add/1 -> Abs/1
  Product1/1 -> B1/1
  Abs/1 -> Product/1, Product1/2

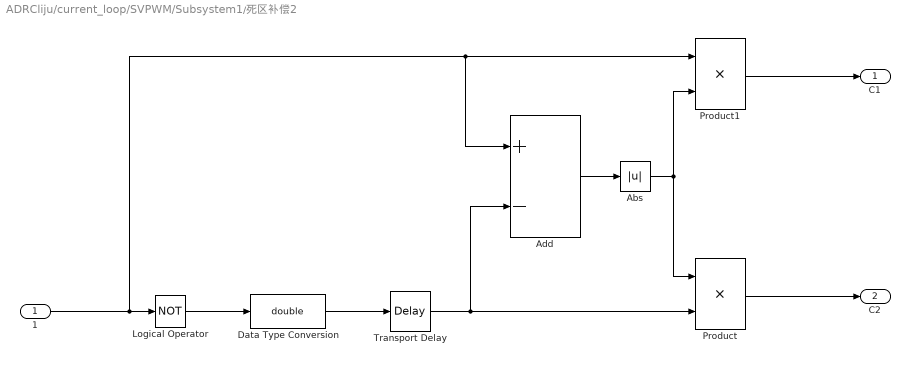
== system ADRCliju/current_loop/SVPWM/Subsystem1/死区补偿2 ==
  1 : Inport
  Abs : Abs  SaturateOnIntegerOverflow=off
  Add : Sum  Inputs=+-
  Data Type Conversion : DataTypeConversion  OutDataTypeStr=double  SaturateOnIntegerOverflow=off  RndMeth=Floor
  Logical Operator : Logic  Operator=NOT  AllPortsSameDT=off  OutDataTypeStr=boolean
  Product : Product
  Product1 : Product
  Transport Delay : TransportDelay  DelayTime=0
  C1 : Outport
  C2 : Outport  Port=2
  wires:
  Abs/1 -> Product1/2, Product/1
  Product1/1 -> C1/1
  Add/1 -> Abs/1
  Product/1 -> C2/1
  Transport Delay/1 -> Product/2, Add/2
  Data Type Conversion/1 -> Transport Delay/1
  Logical Operator/1 -> Data Type Conversion/1
  1/1 -> Logical Operator/1, Add/1, Product1/1

== matlab function ADRCliju/MATLAB Function ==
  settings: updateMethod=DISCRETE
  data: u input; y1k output; y2k output
function [y1k,y2k] = TD(u)
persistent y1k_1 y2k_1
h=0.0015;
delta=1;
if isempty(y1k_1)
    y1k_1=0;
end

if isempty(y2k_1)
    y2k_1=0;
end

y1k=y1k_1+h*y2k_1;

%%%%%%%%%%%%%%%%%%%%%%%%%%%%%%%%%%%%%%%%%%%%%%%hfst计算内容
d=delta*h;
d0=h*d;
y=y1k_1-u+h*y2k_1;
a0=sqrt(d*d+8*delta*abs(y));
a=0;
out1=0;
if abs(y)>d0
    a=y2k_1+(a0-d)/2*sign(y);
end

if abs(y)<=d0
    a=y2k_1+y/h;
end

if abs(a)>d
    out1=-delta*sign(a);
end

if abs(a)<=d
    out1=-delta*a/d;
end
out=out1;
%%%%%%%%%%%%%%%%%%%%%%%%%%%%%%%%%%%%%%%%%%%%

y2k=y2k_1+h*out;

y1k_1=y1k;
y2k_1=y2k;

y1k=y1k;
y2k=y2k;

end

== matlab function ADRCliju/MATLAB Function3 ==
  data: u1 input; y output; u2 input; u3 input
function y = fcn(u1,u2,u3)
y=0;
if u1*u2<0&&abs(u1)>10&&abs(u3)<0.5
    y=1;
end

== matlab function ADRCliju/MATLAB Function1 ==
  settings: updateMethod=DISCRETE  sampleTime=0.001
  data: z3_k output; z2_k output; yk input; z1_k output; uk input
function [z3_k,z2_k,z1_k] = ESO(yk,uk)
%%参数初始化
persistent  z1_k_1 z2_k_1 z3_k_1
bata01=90;
beta02=950;
beta03=8;
%b=5;
h=0.015;
alfa1=0.75;
alfa2=0.75;
delta=1;
fal1=1;
fal2=1;
if isempty(z1_k_1)
    z1_k_1=0;
end
if isempty(z2_k_1)
    z2_k_1=0;
end
if isempty(z3_k_1)
    z3_k_1=0;
end

e1=z1_k_1-yk;
z1_k=z1_k_1+h*(z2_k_1-bata01*e1);
z1_k_1=z1_k; %%迭代更新z1_k_1

%%计算fal函数
if abs(e1)<=delta
    fal1=e1/(delta^(1-alfa1));
end
if abs(e1)>delta
    fal1=(abs(e1))^(alfa1)*sign(e1);
end
if abs(e1)<=delta
    fal2=e1/(delta^(1-alfa2));
end
if abs(e1)>delta
    fal2=(abs(e1))^(alfa2)*sign(e1);
end

z2_k=z2_k_1+h*(z3_k_1-beta02*fal1+uk);
z2_k_1=z2_k;%%迭代更新z2_k_1

z3_k=z3_k_1-h*beta03*fal2;
z3_k_1=z3_k;%%迭代更新z3_k_1

end

== matlab function ADRCliju/MATLAB Function2 ==
  data: e1 input; y output; e2 input
function y =NLSEF(e1,e2)
alfa1=0.75;
alfa2=0.75;
delta=1;
beta1=2;
beta2=1.5;
fal1=1;
fal2=1;

if abs(e1)<=delta
    fal1=e1/(delta^(1-alfa1));
end

if abs(e1)>delta
    fal1=(abs(e1))^(alfa1)*sign(e1);
end

if abs(e2)<=delta
    fal2=e2/(delta^(1-alfa2));
end

if abs(e2)>delta
    fal2=(abs(e2))^(alfa2)*sign(e2);
end

y=beta1*fal1+beta2*fal2;
end

== matlab function ADRCliju/MATLAB Function4 ==
  data: u1 input; y1 output; u2 input; u3 input; y input
function y1 = fcn(u1,u2,u3,y)
y1=0;
if y==1&&u1*u2>0&&abs(u3)>=3
    y1=-1;
end
